simulink model "G474_Hybrid_Flux_Observer"  (R2024b)
settings: Solver=FixedStepDiscrete  StartTime=0.0  StopTime=2  FixedStep=p.Ts  RelTol=1e-3
PostLoadFcn:
  | load_system(fullfile(fileparts(get_param('G474_Hybrid_Flux_Observer','FileName')),'G474_Firmware_PI.slx'));
model workspace (MAT data in the model file):
  observer_input = timeseries
  observer_input.Name = 'Observer input'
  observer_input.DataInfo = tsdata.datametadata
  observer_input.DataInfo.Interpolation = tsdata.interpolation
  observer_input.DataInfo.Interpolation.Fhandle : function handle (value not decoded)
  observer_input.DataInfo.Interpolation.Name = 'linear'
  observer_input.TimeInfo = tsdata.timemetadata
  observer_input.TimeInfo.Length = 40001
  observer_input.TimeInfo.DuplicateTimes = 0
  observer_input.TimeInfo.Time_ = [0 5e-05 0.0001 0.00015 0.0002 0.00025 0.0003 0.00035 0.0004 0.00045 0.0005 0.00055 ... (40001 elements, 40001x1)]
  observer_input.TimeInfo.Initialized = 1
  observer_input.QualityInfo = tsdata.qualmetadata
  observer_input.Data_ = [-0.00508991480522 -0.00644008675394 -0.00779088952634 -0.00914223979853 -0.0104940542129 -0.0118462493831 -0.0131987418994 -0.0145514483336 -0.0159042852446 -0.0172571691829 -0.0186100166963 -0.0199627443347 ... (400010 elements, 40001x10)]
  p.source_commit = 'c43e794924c73d0aec71ddcb6ee14937aa39835e'
  p.Rs = 0.875
  p.Ls = 0.0002
  p.Ld = 0.0002
  p.Lq = 0.0002
  p.Flux = 0.00752
  p.MOTOR_POLES = 14
  p.Ts = 5e-05
  p.Gain = 5000
  p.PLL_BW_Hz = 15
  p.Comp_BW_Hz = 5
  p.PLL_kp = 188.495559215
  p.PLL_ki = 0.444132198049
  p.Comp_Kp = 62.8318530718
  p.Comp_Ki = 0.0493480220054
  p.Comp_Mode = 0
  p.SMO_Kslide = 10
  p.SMO_Boundary = 0.002
  p.V_deadtime = 0.3
  p.current_deadband = 0.01
  p.nominal_bus_voltage = 12
  p.pll_step_limit = 0.157079632679
  p.speed_decimation = 8
  p.speed_filter_old = 0.95
  p.speed_filter_new = 0.05
  s0.psi_s = [0.00756; 0.0002]
  s0.comp_integral = [0; 0]
  s0.theta = 0
  s0.pll_integral = 0
  s0.speed_acc = 0
  s0.speed_count = 0
  s0.speed_hz = 0
  s0.pll_kp = 188.495559215
  s0.pll_ki = 0.444132198049
  s0.pll_ramp_active = 0
  startup_mode = 'aligned'
  truth.time = [0 5e-05 0.0001 0.00015 0.0002 0.00025 0.0003 0.00035 0.0004 0.00045 0.0005 0.00055 ... (40001 elements, 40001x1)]
  truth.theta = [0 0.00785398163397 0.0157079632679 0.0235619449019 0.0314159265359 0.0392699081699 0.0471238898038 0.0549778714378 0.0628318530718 0.0706858347058 0.0785398163397 0.0863937979737 ... (40001 elements, 40001x1)]
  truth.electrical_hz = [25 25 25 25 25 25 25 25 25 25 25 25 ... (40001 elements, 40001x1)]
  truth.active_flux = [0.00752 0.00752 0.00752 0.00752 0.00752 0.00752 0.00752 0.00752 0.00752 0.00752 0.00752 0.00752 ... (40001 elements, 40001x1)]
libraries: G474_Firmware_PI x3
settings Model: Creator=QXZ-030079  LastModifiedBy=QXZ-030079
settings DataIOCC: SignalLogging=off

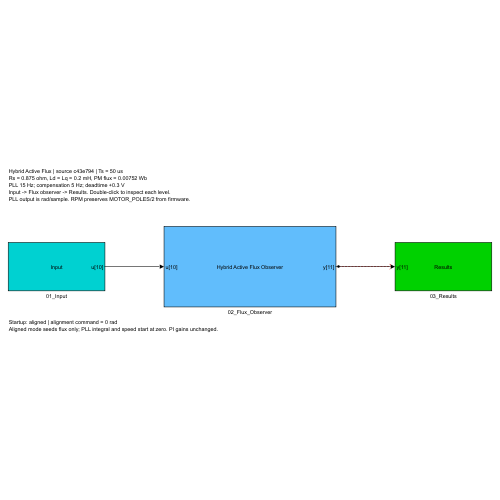
[thumbnail: Simulink's stored preview of the top-level diagram]
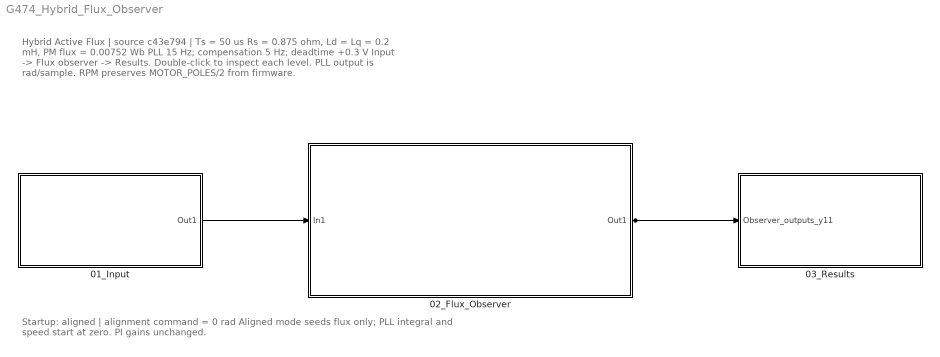
== system G474_Hybrid_Flux_Observer ==
  note: Hybrid Active Flux | source c43e794 | Ts = 50 us
      | Rs = 0.875 ohm, Ld = Lq = 0.2 mH, PM flux = 0.00752 Wb
      | PLL 15 Hz; compensation 5 Hz; deadtime +0.3 V
      | Input -> Flux observer -> Results. Double-click to inspect each level.
      | PLL output is rad/sample. RPM preserves MOTOR_POLES/2 from firmware.
  note: Startup: aligned | alignment command = 0 rad
      | Aligned mode seeds flux only; PLL integral and speed start at zero. PI gains unchanged.
  01_Input : Subsystem
      settings: OpenFcn=open_system(gcb,'force')
      mask Display: disp('Input'); port_label('output',1,'u[10]');
  02_Flux_Observer : Subsystem
      settings: OpenFcn=open_system(gcb,'force')
      mask Display: disp('Hybrid Active Flux Observer'); port_label('input',1,'u[10]'); port_label('output',1,'y[11]');
  03_Results : Subsystem
      settings: OpenFcn=open_system(gcb,'force')
      mask Display: disp('Results'); port_label('input',1,'y[11]');
  wires:
  01_Input/1(Out1) -> 02_Flux_Observer/1(In1)
  02_Flux_Observer/1(Out1) -> 03_Results/1(Observer_outputs_y11)

== system G474_Hybrid_Flux_Observer/01_Input ==
  Inputs : FromWorkspace  VariableName=observer_input  Interpolate=off  OutputAfterFinalValue=Holding final value
  Out1 : Outport
  wires:
  Inputs/1 -> Out1/1

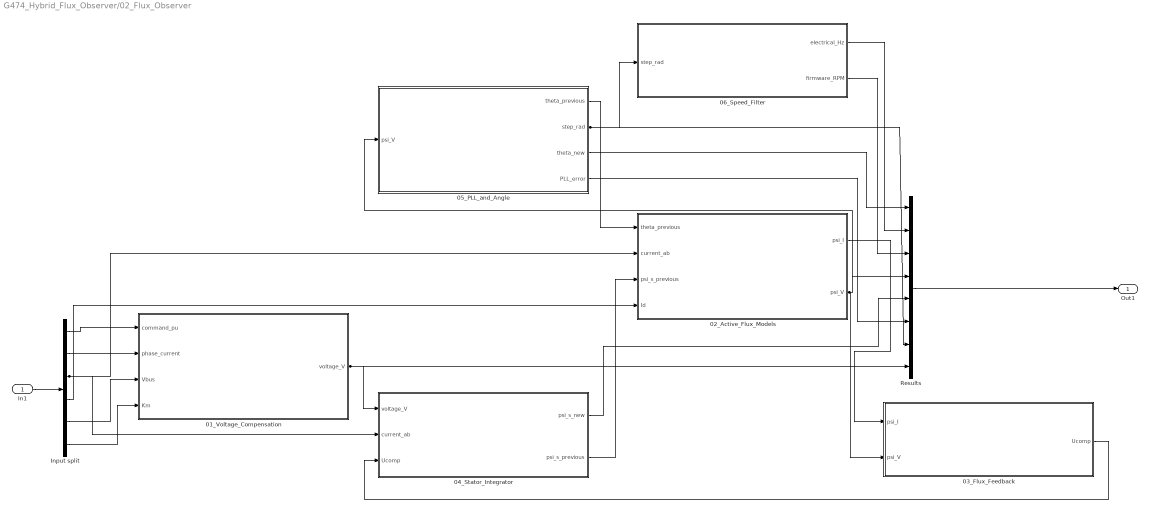
== system G474_Hybrid_Flux_Observer/02_Flux_Observer ==
  In1 : Inport
  01_Voltage_Compensation : Subsystem
      settings: OpenFcn=open_system(gcb,'force')
      mask Display: port_label('input',1,'command_pu');port_label('input',2,'phase_current');port_label('input',3,'Vbus');port_label('input',4,'Km');port_label('output',1,'voltage_V');
  02_Active_Flux_Models : Subsystem
      settings: OpenFcn=open_system(gcb,'force')
      mask Display: port_label('input',1,'theta_previous');port_label('input',2,'current_ab');port_label('input',3,'psi_s_previous');port_label('input',4,'Id');port_label('output',1,'psi_I');port_label('output',2,'psi_V');
  03_Flux_Feedback : Subsystem
      settings: OpenFcn=open_system(gcb,'force')
      mask Display: port_label('input',1,'psi_I');port_label('input',2,'psi_V');port_label('output',1,'Ucomp');
  04_Stator_Integrator : Subsystem
      settings: OpenFcn=open_system(gcb,'force')
      mask Display: port_label('input',1,'voltage_V');port_label('input',2,'current_ab');port_label('input',3,'Ucomp');port_label('output',1,'psi_s_new');port_label('output',2,'psi_s_previous');
  05_PLL_and_Angle : Subsystem
      settings: OpenFcn=open_system(gcb,'force')
      mask Display: port_label('input',1,'psi_V');port_label('output',1,'theta_previous');port_label('output',2,'step_rad');port_label('output',3,'theta_new');port_label('output',4,'PLL_error');
  06_Speed_Filter : Subsystem
      settings: OpenFcn=open_system(gcb,'force')
      mask Display: port_label('input',1,'step_rad');port_label('output',1,'electrical_Hz');port_label('output',2,'firmware_RPM');
  Input split : Demux  Outputs=[2 3 2 1 1 1]
  Results : Mux  Inputs=8
  Out1 : Outport
  wires:
  05_PLL_and_Angle/1(theta_previous) -> 02_Active_Flux_Models/1(theta_previous)
  Input split/2 -> 01_Voltage_Compensation/2(phase_current)
  In1/1 -> Input split/1
  Input split/4 -> 02_Active_Flux_Models/4(Id)
  Input split/1 -> 01_Voltage_Compensation/1(command_pu)
  Input split/3 -> 04_Stator_Integrator/2(current_ab), 02_Active_Flux_Models/2(current_ab)
  Input split/6 -> 01_Voltage_Compensation/4(Km)
  02_Active_Flux_Models/1(psi_I) -> 03_Flux_Feedback/1(psi_I)
  Input split/5 -> 01_Voltage_Compensation/3(Vbus)
  01_Voltage_Compensation/1(voltage_V) -> Results/8, 04_Stator_Integrator/1(voltage_V)
  05_PLL_and_Angle/2(step_rad) -> Results/7, 06_Speed_Filter/1(step_rad)
  05_PLL_and_Angle/3(theta_new) -> Results/1
  05_PLL_and_Angle/4(PLL_error) -> Results/6
  04_Stator_Integrator/1(psi_s_new) -> Results/5
  04_Stator_Integrator/2(psi_s_previous) -> 02_Active_Flux_Models/3(psi_s_previous)
  Results/1 -> Out1/1
  06_Speed_Filter/1(electrical_Hz) -> Results/2
  06_Speed_Filter/2(firmware_RPM) -> Results/3
  02_Active_Flux_Models/2(psi_V) -> 03_Flux_Feedback/2(psi_V), Results/4, 05_PLL_and_Angle/1(psi_V)
  03_Flux_Feedback/1(Ucomp) -> 04_Stator_Integrator/3(Ucomp)

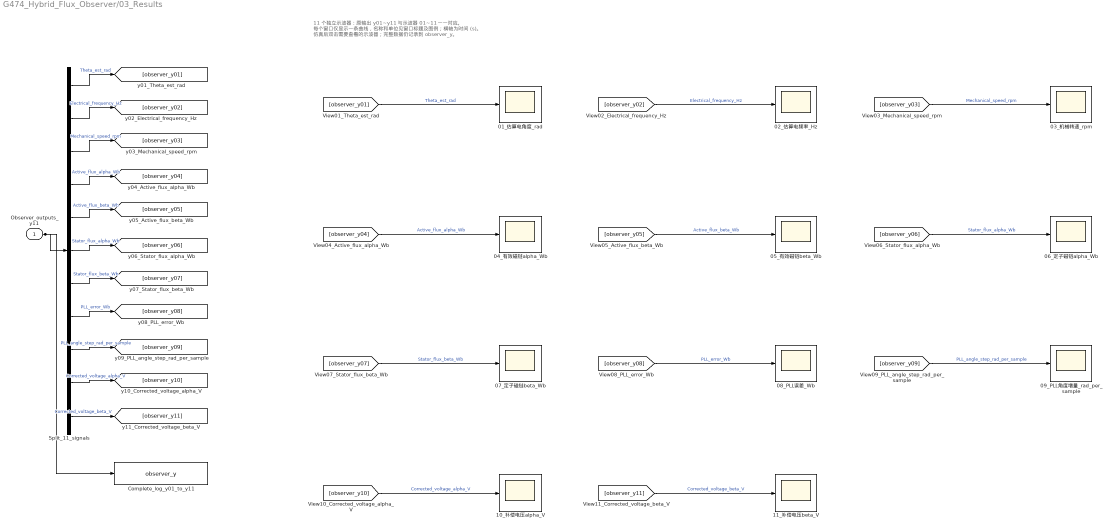
== system G474_Hybrid_Flux_Observer/03_Results ==
  note: 11 个独立示波器：原输出 y01~y11 与示波器 01~11 一一对应。
      | 每个窗口仅显示一条曲线，名称和单位见窗口标题及图例；横轴为时间 (s)。
      | 仿真后双击需要查看的示波器；完整数据仍记录到 observer_y。
  Observer_outputs_y11 : Inport
  01_估算电角度_rad : Scope
  02_估算电频率_Hz : Scope
  03_机械转速_rpm : Scope
  04_有效磁链alpha_Wb : Scope
  05_有效磁链beta_Wb : Scope
  06_定子磁链alpha_Wb : Scope
  07_定子磁链beta_Wb : Scope
  08_PLL误差_Wb : Scope
  09_PLL角度增量_rad_per_sample : Scope
  10_补偿电压alpha_V : Scope
  11_补偿电压beta_V : Scope
  Complete_log_y01_to_y11 : ToWorkspace  VariableName=observer_y  SaveFormat=Timeseries  SampleTime=-1
  Split_11_signals : Demux  Outputs=11
  wires:
  Observer_outputs_y11/1 -> Split_11_signals/1, Complete_log_y01_to_y11/1
  Split_11_signals/1 -> [observer_y01]  "Theta_est_rad"
  [observer_y01] -> 01_估算电角度_rad/1  "Theta_est_rad"
  Split_11_signals/2 -> [observer_y02]  "Electrical_frequency_Hz"
  [observer_y02] -> 02_估算电频率_Hz/1  "Electrical_frequency_Hz"
  Split_11_signals/3 -> [observer_y03]  "Mechanical_speed_rpm"
  [observer_y03] -> 03_机械转速_rpm/1  "Mechanical_speed_rpm"
  Split_11_signals/4 -> [observer_y04]  "Active_flux_alpha_Wb"
  [observer_y04] -> 04_有效磁链alpha_Wb/1  "Active_flux_alpha_Wb"
  Split_11_signals/5 -> [observer_y05]  "Active_flux_beta_Wb"
  [observer_y05] -> 05_有效磁链beta_Wb/1  "Active_flux_beta_Wb"
  Split_11_signals/6 -> [observer_y06]  "Stator_flux_alpha_Wb"
  [observer_y06] -> 06_定子磁链alpha_Wb/1  "Stator_flux_alpha_Wb"
  Split_11_signals/7 -> [observer_y07]  "Stator_flux_beta_Wb"
  [observer_y07] -> 07_定子磁链beta_Wb/1  "Stator_flux_beta_Wb"
  Split_11_signals/8 -> [observer_y08]  "PLL_error_Wb"
  [observer_y08] -> 08_PLL误差_Wb/1  "PLL_error_Wb"
  Split_11_signals/9 -> [observer_y09]  "PLL_angle_step_rad_per_sample"
  [observer_y09] -> 09_PLL角度增量_rad_per_sample/1  "PLL_angle_step_rad_per_sample"
  Split_11_signals/10 -> [observer_y10]  "Corrected_voltage_alpha_V"
  [observer_y10] -> 10_补偿电压alpha_V/1  "Corrected_voltage_alpha_V"
  Split_11_signals/11 -> [observer_y11]  "Corrected_voltage_beta_V"
  [observer_y11] -> 11_补偿电压beta_V/1  "Corrected_voltage_beta_V"

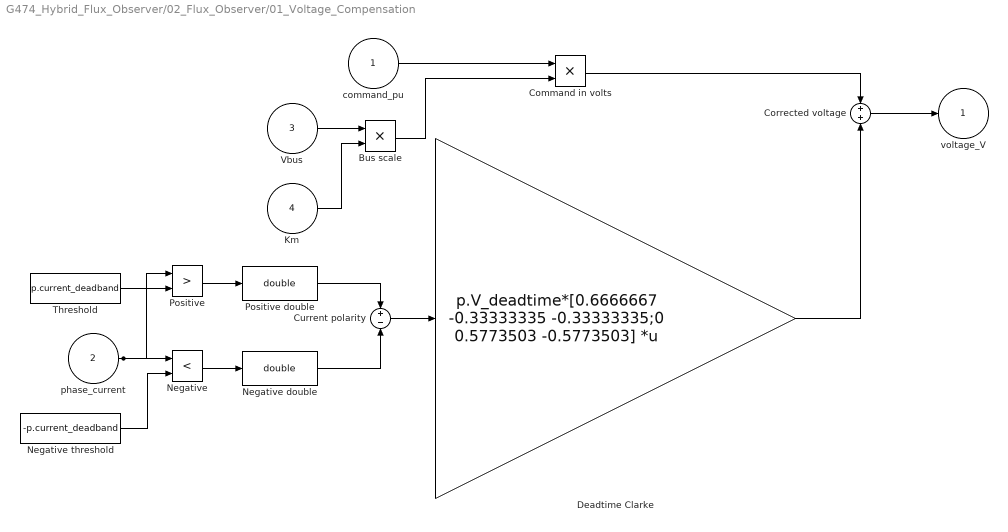
== system G474_Hybrid_Flux_Observer/02_Flux_Observer/01_Voltage_Compensation ==
  command_pu : Inport
  phase_current : Inport  Port=2
  Vbus : Inport  Port=3
  Km : Inport  Port=4
  Bus scale : Product  Inputs=**
  Command in volts : Product  Inputs=**
  Corrected voltage : Sum
  Current polarity : Sum  Inputs=+-
  Deadtime Clarke : Gain  Gain=p.V_deadtime*[0.6666667 -0.33333335 -0.33333335;0 0.5773503 -0.5773503]  Multiplication=Matrix(K*u)
  Negative : RelationalOperator  Operator=<  OutDataTypeStr=boolean  RndMeth=Simplest  InputSameDT=off
  Negative double : DataTypeConversion  OutDataTypeStr=double  SaturateOnIntegerOverflow=off  RndMeth=Floor
  Negative threshold : Constant  Value=-p.current_deadband
  Positive : RelationalOperator  Operator=>  OutDataTypeStr=boolean  RndMeth=Simplest  InputSameDT=off
  Positive double : DataTypeConversion  OutDataTypeStr=double  SaturateOnIntegerOverflow=off  RndMeth=Floor
  Threshold : Constant  Value=p.current_deadband
  voltage_V : Outport
  wires:
  Threshold/1 -> Positive/2
  Positive/1 -> Positive double/1
  phase_current/1 -> Positive/1, Negative/1
  Km/1 -> Bus scale/2
  Negative threshold/1 -> Negative/2
  Positive double/1 -> Current polarity/1
  Negative/1 -> Negative double/1
  Negative double/1 -> Current polarity/2
  Vbus/1 -> Bus scale/1
  command_pu/1 -> Command in volts/1
  Bus scale/1 -> Command in volts/2
  Current polarity/1 -> Deadtime Clarke/1
  Command in volts/1 -> Corrected voltage/1
  Deadtime Clarke/1 -> Corrected voltage/2
  Corrected voltage/1 -> voltage_V/1

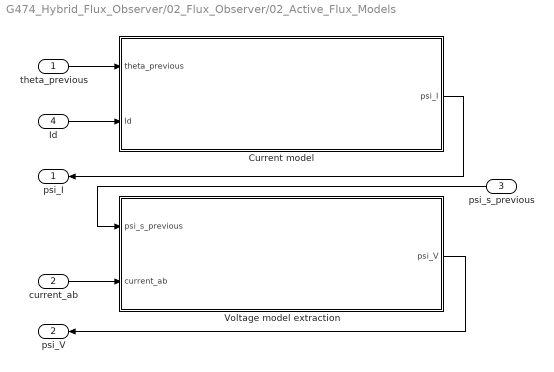
== system G474_Hybrid_Flux_Observer/02_Flux_Observer/02_Active_Flux_Models ==
  theta_previous : Inport
  current_ab : Inport  Port=2
  psi_s_previous : Inport  Port=3
  Id : Inport  Port=4
  Current model : Subsystem
      settings: OpenFcn=open_system(gcb,'force')
      mask Display: port_label('input',1,'theta_previous');port_label('input',2,'Id');port_label('output',1,'psi_I');
  Voltage model extraction : Subsystem
      settings: OpenFcn=open_system(gcb,'force')
      mask Display: port_label('input',1,'psi_s_previous');port_label('input',2,'current_ab');port_label('output',1,'psi_V');
  psi_I : Outport
  psi_V : Outport  Port=2
  wires:
  theta_previous/1 -> Current model/1(theta_previous)
  Voltage model extraction/1(psi_V) -> psi_V/1
  Id/1 -> Current model/2(Id)
  current_ab/1 -> Voltage model extraction/2(current_ab)
  Current model/1(psi_I) -> psi_I/1
  psi_s_previous/1 -> Voltage model extraction/1(psi_s_previous)

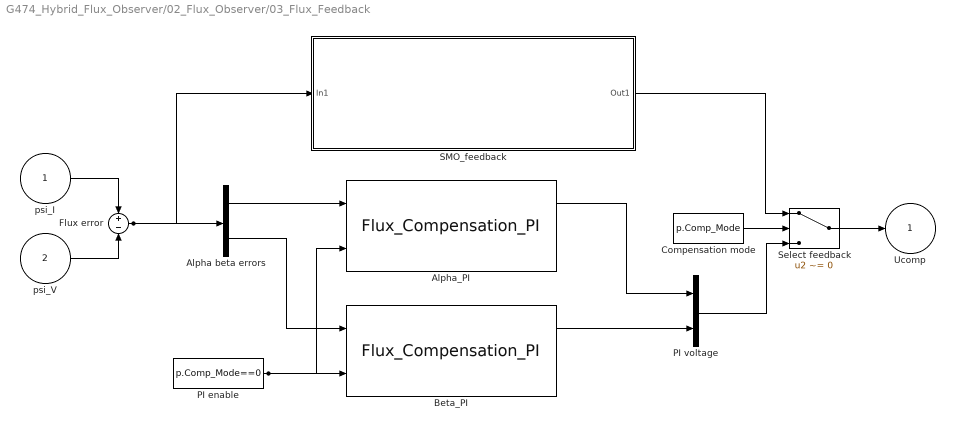
== system G474_Hybrid_Flux_Observer/02_Flux_Observer/03_Flux_Feedback ==
  psi_I : Inport
  psi_V : Inport  Port=2
  Alpha beta errors : Demux  Outputs=2
  Alpha_PI : G474_Firmware_PI/Flux_Compensation_PI  Kp=p.Comp_Kp  Ki=p.Comp_Ki  Ts=p.Ts
  Beta_PI : G474_Firmware_PI/Flux_Compensation_PI  Kp=p.Comp_Kp  Ki=p.Comp_Ki  Ts=p.Ts
  Compensation mode : Constant  Value=p.Comp_Mode
  Flux error : Sum  Inputs=+-
  PI enable : Constant  Value=p.Comp_Mode==0
  PI voltage : Mux  Inputs=2
  SMO_feedback : Subsystem
      settings: OpenFcn=open_system(gcb,'force')
      mask Display: port_label('input',1,'In1');port_label('output',1,'Out1');
  Select feedback : Switch  Criteria=u2 ~= 0  SaturateOnIntegerOverflow=off  InputSameDT=off
  Ucomp : Outport
  wires:
  Alpha beta errors/1 -> Alpha_PI/1
  PI voltage/1 -> Select feedback/3
  psi_I/1 -> Flux error/1
  Flux error/1 -> SMO_feedback/1(In1), Alpha beta errors/1
  psi_V/1 -> Flux error/2
  Alpha beta errors/2 -> Beta_PI/1
  PI enable/1 -> Alpha_PI/2, Beta_PI/2
  SMO_feedback/1(Out1) -> Select feedback/1
  Alpha_PI/1 -> PI voltage/1
  Beta_PI/1 -> PI voltage/2
  Compensation mode/1 -> Select feedback/2
  Select feedback/1 -> Ucomp/1

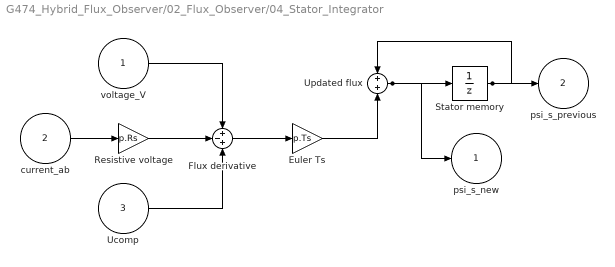
== system G474_Hybrid_Flux_Observer/02_Flux_Observer/04_Stator_Integrator ==
  voltage_V : Inport
  current_ab : Inport  Port=2
  Ucomp : Inport  Port=3
  Euler Ts : Gain  Gain=p.Ts
  Flux derivative : Sum  Inputs=+-+
  Resistive voltage : Gain  Gain=p.Rs
  Stator memory : UnitDelay  InitialCondition=s0.psi_s  SampleTime=p.Ts  HasFrameUpgradeWarning=on
  Updated flux : Sum
  psi_s_new : Outport
  psi_s_previous : Outport  Port=2
  wires:
  current_ab/1 -> Resistive voltage/1
  Ucomp/1 -> Flux derivative/3
  voltage_V/1 -> Flux derivative/1
  Stator memory/1 -> Updated flux/1, psi_s_previous/1
  Resistive voltage/1 -> Flux derivative/2
  Flux derivative/1 -> Euler Ts/1
  Updated flux/1 -> psi_s_new/1, Stator memory/1
  Euler Ts/1 -> Updated flux/2

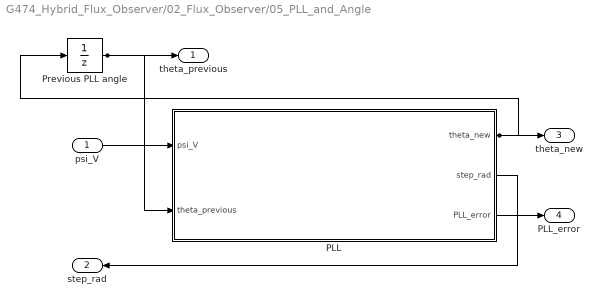
== system G474_Hybrid_Flux_Observer/02_Flux_Observer/05_PLL_and_Angle ==
  psi_V : Inport
  PLL : Subsystem
      settings: OpenFcn=open_system(gcb,'force')
      mask Display: port_label('input',1,'psi_V');port_label('input',2,'theta_previous');port_label('output',1,'theta_new');port_label('output',2,'step_rad');port_label('output',3,'PLL_error');
  Previous PLL angle : UnitDelay  InitialCondition=s0.theta  SampleTime=p.Ts  HasFrameUpgradeWarning=on
  theta_previous : Outport
  step_rad : Outport  Port=2
  theta_new : Outport  Port=3
  PLL_error : Outport  Port=4
  wires:
  PLL/3(PLL_error) -> PLL_error/1
  Previous PLL angle/1 -> PLL/2(theta_previous), theta_previous/1
  PLL/1(theta_new) -> Previous PLL angle/1, theta_new/1
  psi_V/1 -> PLL/1(psi_V)
  PLL/2(step_rad) -> step_rad/1

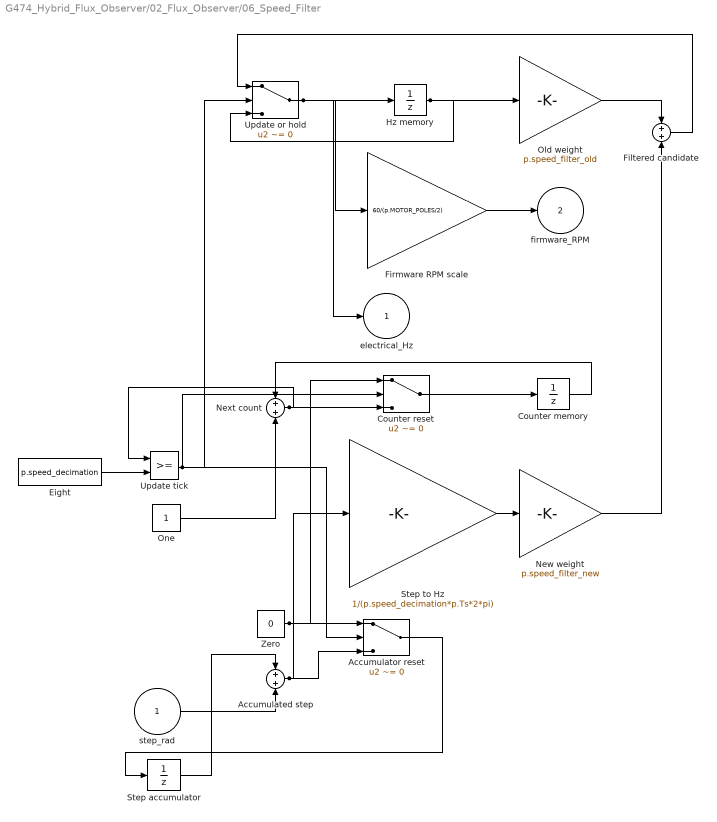
== system G474_Hybrid_Flux_Observer/02_Flux_Observer/06_Speed_Filter ==
  step_rad : Inport
  Accumulated step : Sum
  Accumulator reset : Switch  Criteria=u2 ~= 0  SaturateOnIntegerOverflow=off  InputSameDT=off
  Counter memory : UnitDelay  SampleTime=p.Ts  HasFrameUpgradeWarning=on
  Counter reset : Switch  Criteria=u2 ~= 0  SaturateOnIntegerOverflow=off  InputSameDT=off
  Eight : Constant  Value=p.speed_decimation
  Filtered candidate : Sum
  Firmware RPM scale : Gain  Gain=60/(p.MOTOR_POLES/2)
  Hz memory : UnitDelay  SampleTime=p.Ts  HasFrameUpgradeWarning=on
  New weight : Gain  Gain=p.speed_filter_new
  Next count : Sum
  Old weight : Gain  Gain=p.speed_filter_old
  One : Constant
  Step accumulator : UnitDelay  SampleTime=p.Ts  HasFrameUpgradeWarning=on
  Step to Hz : Gain  Gain=1/(p.speed_decimation*p.Ts*2*pi)
  Update or hold : Switch  Criteria=u2 ~= 0  SaturateOnIntegerOverflow=off  InputSameDT=off
  Update tick : RelationalOperator  OutDataTypeStr=boolean  RndMeth=Simplest  InputSameDT=off
  Zero : Constant  Value=0
  electrical_Hz : Outport
  firmware_RPM : Outport  Port=2
  wires:
  Accumulator reset/1 -> Step accumulator/1
  Zero/1 -> Counter reset/1, Accumulator reset/1
  One/1 -> Next count/2
  Eight/1 -> Update tick/2
  Next count/1 -> Counter reset/3, Update tick/1
  Update tick/1 -> Counter reset/2, Accumulator reset/2, Update or hold/2
  Firmware RPM scale/1 -> firmware_RPM/1
  step_rad/1 -> Accumulated step/2
  Step accumulator/1 -> Accumulated step/1
  Step to Hz/1 -> New weight/1
  Update or hold/1 -> Hz memory/1, electrical_Hz/1, Firmware RPM scale/1
  Accumulated step/1 -> Accumulator reset/3, Step to Hz/1
  Hz memory/1 -> Update or hold/3, Old weight/1
  Counter reset/1 -> Counter memory/1
  Old weight/1 -> Filtered candidate/1
  Counter memory/1 -> Next count/1
  New weight/1 -> Filtered candidate/2
  Filtered candidate/1 -> Update or hold/1

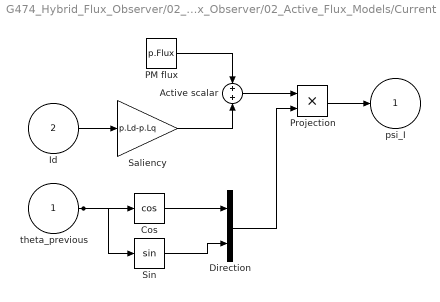
== system G474_Hybrid_Flux_Observer/02_Flux_Observer/02_Active_Flux_Models/Current model ==
  theta_previous : Inport
  Id : Inport  Port=2
  Active scalar : Sum
  Cos : Trigonometry  Operator=cos
  Direction : Mux  Inputs=2
  PM flux : Constant  Value=p.Flux
  Projection : Product  Inputs=**
  Saliency : Gain  Gain=p.Ld-p.Lq
  Sin : Trigonometry
  psi_I : Outport
  wires:
  Id/1 -> Saliency/1
  Direction/1 -> Projection/2
  theta_previous/1 -> Sin/1, Cos/1
  PM flux/1 -> Active scalar/1
  Saliency/1 -> Active scalar/2
  Cos/1 -> Direction/1
  Active scalar/1 -> Projection/1
  Sin/1 -> Direction/2
  Projection/1 -> psi_I/1

== system G474_Hybrid_Flux_Observer/02_Flux_Observer/02_Active_Flux_Models/Voltage model extraction ==
  psi_s_previous : Inport
  current_ab : Inport  Port=2
  Active flux : Sum  Inputs=+-
  Inductive flux : Gain  Gain=p.Lq
  psi_V : Outport
  wires:
  current_ab/1 -> Inductive flux/1
  psi_s_previous/1 -> Active flux/1
  Inductive flux/1 -> Active flux/2
  Active flux/1 -> psi_V/1

== system G474_Hybrid_Flux_Observer/02_Flux_Observer/03_Flux_Feedback/SMO_feedback ==
  In1 : Inport
  Boundary normalization : Gain  Gain=1/p.SMO_Boundary
  Boundary saturation : Saturate  UpperLimit=1  LowerLimit=-1
  Sliding gain : Gain  Gain=p.SMO_Kslide
  Out1 : Outport
  wires:
  Boundary normalization/1 -> Boundary saturation/1
  In1/1 -> Boundary normalization/1
  Boundary saturation/1 -> Sliding gain/1
  Sliding gain/1 -> Out1/1

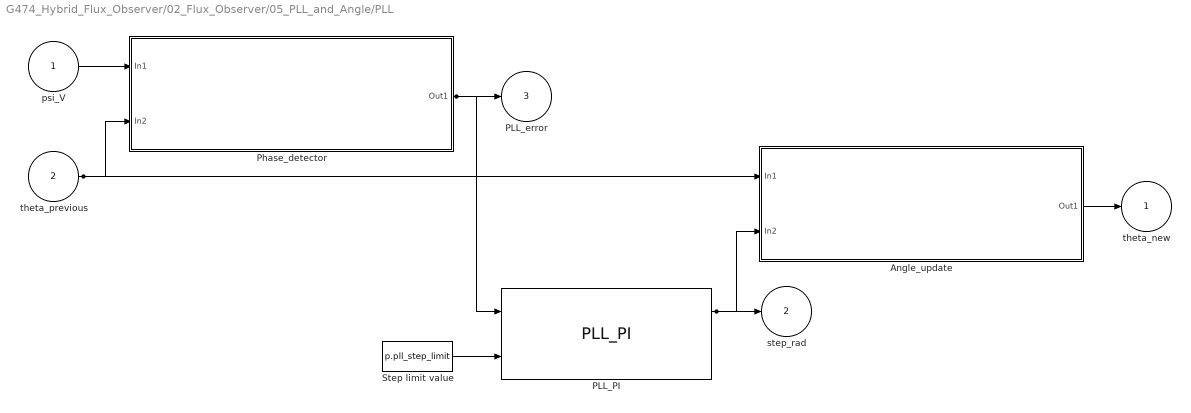
== system G474_Hybrid_Flux_Observer/02_Flux_Observer/05_PLL_and_Angle/PLL ==
  psi_V : Inport
  theta_previous : Inport  Port=2
  Angle_update : Subsystem
      settings: OpenFcn=open_system(gcb,'force')
      mask Display: port_label('input',1,'In1');port_label('input',2,'In2');port_label('output',1,'Out1');
  PLL_PI : G474_Firmware_PI/PLL_PI  Kp=p.PLL_kp  Ki=p.PLL_ki  Ts=p.Ts
  Phase_detector : Subsystem
      settings: OpenFcn=open_system(gcb,'force')
      mask Display: port_label('input',1,'In1');port_label('input',2,'In2');port_label('output',1,'Out1');
  Step limit value : Constant  Value=p.pll_step_limit
  theta_new : Outport
  step_rad : Outport  Port=2
  PLL_error : Outport  Port=3
  wires:
  psi_V/1 -> Phase_detector/1(In1)
  theta_previous/1 -> Phase_detector/2(In2), Angle_update/1(In1)
  PLL_PI/1 -> step_rad/1, Angle_update/2(In2)
  Phase_detector/1(Out1) -> PLL_PI/1, PLL_error/1
  Step limit value/1 -> PLL_PI/2
  Angle_update/1(Out1) -> theta_new/1

== system G474_Hybrid_Flux_Observer/02_Flux_Observer/05_PLL_and_Angle/PLL/Angle_update ==
  In1 : Inport
  In2 : Inport  Port=2
  Angle update : Sum
  Two pi : Constant  Value=2*pi
  Wrap 2pi : Math  Operator=mod
  Out1 : Outport
  wires:
  Two pi/1 -> Wrap 2pi/2
  In2/1 -> Angle update/2
  Angle update/1 -> Wrap 2pi/1
  Wrap 2pi/1 -> Out1/1
  In1/1 -> Angle update/1

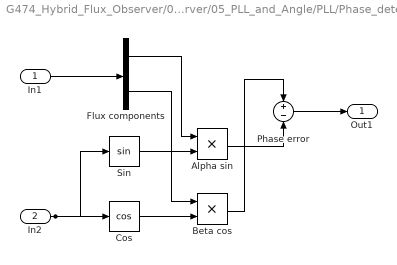
== system G474_Hybrid_Flux_Observer/02_Flux_Observer/05_PLL_and_Angle/PLL/Phase_detector ==
  In1 : Inport
  In2 : Inport  Port=2
  Alpha sin : Product  Inputs=**
  Beta cos : Product  Inputs=**
  Cos : Trigonometry  Operator=cos
  Flux components : Demux  Outputs=2
  Phase error : Sum  Inputs=+-
  Sin : Trigonometry
  Out1 : Outport
  wires:
  In1/1 -> Flux components/1
  Beta cos/1 -> Phase error/1
  In2/1 -> Sin/1, Cos/1
  Sin/1 -> Alpha sin/2
  Flux components/1 -> Alpha sin/1
  Flux components/2 -> Beta cos/1
  Alpha sin/1 -> Phase error/2
  Cos/1 -> Beta cos/2
  Phase error/1 -> Out1/1
